simulink model "F1_Simulator"  (R2026a)
settings: Solver=VariableStepAuto  StopTime=260  MaxStep=0.01
values from neighbouring files (symbols this model uses):
  C = [C; C(1,:)]    [f1_corner_map.m]    (also in f1_lateral_tire_table.m = 1.3; f1_sector_map.m = C([true; hypot(diff(C(:,1)), diff(C(:,2))) > 1e-6], :); f1_sensitivity_sweep.m = {; f1_telemetry.m = C([true; hypot(diff(C(:,1)), diff(C(:,2))) > 1e-6], :))
  m = sU >= d0 & sU <= d1    [f1_corner_map.m]    (also in f1_sector_map.m = dC >= edM(k) & dC <= edM(k+1); f1_speed_profile.m = veh.m)
  normalX = -tangentY    [f1_finish_line_params.m]
  normalY = tangentX    [f1_finish_line_params.m]
  s = cumtrapz(tg, v)    [f1_internal_states.m]    (also in f1_track_animation.m = [0; cumsum(hypot(diff(x), diff(y)))]; f1_track_curvature.m = s_all(keepIdx))
  startX = track(1,1)    [f1_finish_line_params.m]
  startY = track(1,2)    [f1_finish_line_params.m]
  tangentX = dirVec(1)    [f1_finish_line_params.m]
  tangentY = dirVec(2)    [f1_finish_line_params.m]
  trackPsi = psi(idx)    [f1_load_raceline.m]    (also in f1_track_curvature.m = atan2(gradient(trackY), gradient(trackX)))
  trackVref = min(trackVref, vf)    [f1_speed_profile.m]
  trackX = x0    [f1_load_raceline.m]    (also in f1_track_curvature.m = x; silverstone_curvature.mat = [-563.032417564 -561.782952087 -560.539483404 -559.300900612)
  trackY = y0    [f1_load_raceline.m]    (also in f1_track_curvature.m = y; silverstone_curvature.mat = [-515.713759288 -514.151171661 -512.584488731 -511.014091481)
undefined symbols (not defined in the file or in its folder): fp_brk_bore, fp_brk_front, fp_brk_maxT, fp_brk_mu_k, fp_brk_pads, fp_brk_Rm, fp_CdA_corner, fp_CdA_straight, fp_eta_tr, fp_gears, fp_h_cg, fp_mu_brake, fp_mu_pk, fp_mu_trac, fp_N_diff, fp_rho, fp_rpm_dn, fp_rpm_lim_end, fp_rpm_lim_ini, fp_rpm_up, fp_track, pwr, veh
libraries: vehdynlibtire x4, autolibsharedcoupling x3, simulink x1, vehdynlibdriver x1, autolibsharedtransfixedgear x1, autolibshareddiff x1, autolibsharedmappedengines x1, autolibshared x1
(part 5 of 5)

== matlab function F1_Simulator/Vehicle Dynamics/Subsystem1/MATLAB Function3 ==
  data: TrqCmd_req input; TrqCmd output; EngSpd input; FzFL input; FzFR input; FzRL input; FzRR input; Re input; Gear input; fp_N_diff parameter; fp_eta_tr parameter; fp_gears parameter; fp_h_cg parameter; fp_mu_pk parameter; fp_mu_trac parameter; fp_rpm_lim_end parameter; fp_rpm_lim_ini parameter; fp_track parameter
function TrqCmd = f1_engine_cmd(TrqCmd_req, EngSpd, FzFL, FzFR, FzRL, FzRR, Re, Gear, fp_N_diff, fp_eta_tr, fp_gears, fp_h_cg, fp_mu_pk, fp_mu_trac, fp_rpm_lim_end, fp_rpm_lim_ini, fp_track)
% f1_engine_cmd  Engine torque command with (a) a grip limit and (b) a rev
% limiter. No states or loops: it cannot oscillate.
%
% (a) With an OPEN DIFFERENTIAL both wheels get the SAME torque, so the axle
%     can only push what the WEAKEST wheel holds:
%         T_axle <= 2*mu*min(FzRL, FzRR)*Re
%     (the inner wheel unloads in a corner, spins alone and the engine runs
%     into the rev limit). It is converted to ENGINE torque by dividing by the
%     total engine->axle ratio:
%       N_total = N_gear * N_diff * efficiency
%     The cut is made at the source (engine), not at the wheels, because
%     clipping the torque between two Torsional Compliance blocks leaves the
%     spring twisting without limit.
% (b) Above rpm_ini the torque ramps linearly down to 0 at rpm_fin. Without
%     it the engine map (held constant past 16000 rpm) would keep delivering
%     maximum torque at absurd speeds.
%
% Inputs
%   TrqCmd_req : torque requested from the engine [N*m] (the map reaches ~682)
%   EngSpd     : engine speed [rad/s]  (EngSpd output of the transmission)
%   FzFL..FzRR : vertical load of each wheel [N]. The rear ones limit the
%                torque; all 4 estimate how much grip the corner already uses
%                (friction circle)
%   Re         : effective wheel radius [m]
%   Gear       : engaged gear (2..8), from f1_shift_logic
% Output
%   TrqCmd     : command to the Mapped SI Engine [N*m]
%
% FRICTION CIRCLE: the grip available to push is what the tire has left after
% the lateral grip the corner already uses:
%     mu_x = min(mu, sqrt(mu_pk^2 - mu_y^2))
% with mu_y = Fy/sum(Fz) = |sum(Fz right) - sum(Fz left)| * track / (2*h_cg*sum(Fz))
% (the lateral load transfer measures the lateral force the car is making).
% With useFC = false the plain limit is recovered (mu_x = mu). No states or
% loops. If the torque oscillated, filter mu_y with a Transfer Fcn
% 1/(0.05 s + 1) in Simulink before it enters here.
%
% 7-SPEED GEARBOX (gears 2..8): ratio of the engaged gear = N vector of the
% transmission (at Re = 0.3515 m, from real telemetry).
%
% All shared values come from f1_vehicle_params.m through Parameter data
% (fp_*): change them there, not here.

Gvec     = [2 3 4 5 6 7 8];
Nvec     = fp_gears;
N_marcha = interp1(Gvec, Nvec, min(max(Gear, 2), 8), 'nearest');
N_diff   = fp_N_diff;          % final drive of the Active Differential
eta      = fp_eta_tr;          % transmission efficiency
mu       = fp_mu_trac;         % grip used by the limiter (real peak ~1.7)
rpm_ini  = fp_rpm_lim_ini;     % starts cutting
rpm_fin  = fp_rpm_lim_end;     % full cut
useFC    = true;               % friction circle (false = plain limit)
mu_pk    = fp_mu_pk;           % tire peak (Cy tables: 1.7 front / 1.8 rear)
mu_min   = 0.3;                % floor of mu_x: the push never goes fully to zero
track    = fp_track;           % [m] track (veh.track_f/r)
h_cg     = fp_h_cg;            % [m] = veh.cg_height (same h as the Vehicle Body load transfer)

% grip available to push (friction circle)
if useFC
    FzT  = max(FzFL + FzFR + FzRL + FzRR, 1);
    mu_y = min(abs((FzFR + FzRR) - (FzFL + FzRL)) * track / (2 * h_cg * FzT), mu_pk);
    mu_x = min(mu, max(sqrt(mu_pk^2 - mu_y^2), mu_min));
else
    mu_x = mu;
end

% (a) grip limit, as engine torque
Fz_w     = max(min(FzRL, FzRR), 0);   % weakest wheel (open differential)
Tmax_eje = 2 * mu_x * Fz_w * Re;
T_grip   = Tmax_eje / (N_marcha * N_diff * eta);

% (b) rev limiter
rpm = EngSpd * 30 / pi;
f   = min(1, max(0, (rpm_fin - rpm) / (rpm_fin - rpm_ini)));

TrqCmd = max(0, min(TrqCmd_req, T_grip)) * f;
end

== matlab function F1_Simulator/Pilot/MATLAB Function2 ==
  data: AccelCmd input; TrqCmd_req output; DecelCmd input; FzFL input; FzFR input; FzRL input; FzRR input; Re input; PrsFL output; PrsFR output; PrsRL output; PrsRR output; fp_brk_Rm parameter; fp_brk_bore parameter; fp_brk_front parameter; fp_brk_maxT parameter; fp_brk_mu_k parameter; fp_brk_pads parameter; fp_h_cg parameter; fp_mu_brake parameter; fp_mu_pk parameter; fp_track parameter
function [TrqCmd_req, PrsFL, PrsFR, PrsRL, PrsRR] = f1_pedals_to_cmd(AccelCmd, DecelCmd, FzFL, FzFR, FzRL, FzRR, Re, fp_brk_Rm, fp_brk_bore, fp_brk_front, fp_brk_maxT, fp_brk_mu_k, fp_brk_pads, fp_h_cg, fp_mu_brake, fp_mu_pk, fp_track)
% f1_pedals_to_cmd  Converts AccelCmd and DecelCmd from the Predictive Driver
% (0 to 1) into:
%   - TrqCmd_req : torque requested from the engine (goes to f1_engine_cmd,
%                  which applies the grip limit and the rev limit)
%   - PrsXX      : brake pressure of each wheel [Pa] (BrkPrs input of each
%                  Combined Slip Wheel with Brake type = Disc)
%
% The brake output is PRESSURE, not torque, because the BrkPrs port of the
% tire asks for it.
%
% Disc brake torque of the block (MathWorks documentation):
%     T = mu_kinetic * P * (pi*disk_abore^2/4) * Rm * num_pads
% so   P = T / Kdisc   with   Kdisc = mu_kinetic*pi*disk_abore^2/4*Rm*num_pads
% IMPORTANT: the disc parameters (brk.* in f1_vehicle_params.m) must be EQUAL
% to those of the Disc brake of the 4 tires.
%
% The brake is grip-limited in open loop (no feedback, cannot oscillate):
%     T_wheel <= mu_b * Fz_wheel * Re
%
% Inputs
%   AccelCmd, DecelCmd : normalized outputs of the Predictive Driver
%   FzFL..FzRR         : vertical load of each wheel [N]
%   Re                 : effective radius [m]
%
% FRICTION CIRCLE: when braking in a corner the tire is already spending
% lateral grip, so the brake limit drops:
%     mu_x = min(mu_b, sqrt(mu_pk^2 - mu_y^2)),   mu_y = Fy/sum(Fz)
% (mu_y is estimated from the lateral load transfer). With useFC = false the
% plain limit is recovered (mu_x = mu_b). No states.
%
% Shared values come from f1_vehicle_params.m through Parameter data (fp_*).

% --- powertrain and brake parameters ---
maxThrottleTrq = 682;            % N*m, maximum engine torque (end of the map)
maxBrakeTrq    = fp_brk_maxT;    % N*m, TOTAL brake torque on the 4 wheels
frontBias      = fp_brk_front;   % fraction of the braking on the front axle
mu_b           = fp_mu_brake;    % grip used by the brake limiter
useFC          = true;           % friction circle (false = plain limit)
mu_pk          = fp_mu_pk;       % tire peak
mu_min         = 0.3;            % floor of mu_x
track          = fp_track;       % [m] track
h_cg           = fp_h_cg;        % [m] = veh.cg_height (same h as the Vehicle Body load transfer)

% --- disc parameters (equal to those of each wheel block) ---
mu_k       = fp_brk_mu_k;        % mu_kinetic
disk_abore = fp_brk_bore;        % m
Rm         = fp_brk_Rm;          % m
num_pads   = fp_brk_pads;
Kdisc = mu_k * pi * disk_abore^2 / 4 * Rm * num_pads;   % N*m per Pa

acc = min(1, max(0, AccelCmd));
dec = min(1, max(0, DecelCmd));

% Throttle: fades out continuously when braking (no hard switch, to avoid
% zero crossings)
TrqCmd_req = maxThrottleTrq * acc * max(0, 1 - 5*dec);

% Brake: torque demand per wheel according to the split
demF = dec * maxBrakeTrq * frontBias / 2;          % each front wheel
demR = dec * maxBrakeTrq * (1 - frontBias) / 2;    % each rear wheel

% Grip available for braking (friction circle)
if useFC
    FzT  = max(FzFL + FzFR + FzRL + FzRR, 1);
    mu_y = min(abs((FzFR + FzRR) - (FzFL + FzRL)) * track / (2 * h_cg * FzT), mu_pk);
    mu_x = min(mu_b, max(sqrt(mu_pk^2 - mu_y^2), mu_min));
else
    mu_x = mu_b;
end

% Grip limit per wheel (as torque)
TFL = min(demF, mu_x * max(FzFL, 0) * Re);
TFR = min(demF, mu_x * max(FzFR, 0) * Re);
TRL = min(demR, mu_x * max(FzRL, 0) * Re);
TRR = min(demR, mu_x * max(FzRR, 0) * Re);

% Torque to pressure [Pa]
PrsFL = TFL / Kdisc;
PrsFR = TFR / Kdisc;
PrsRL = TRL / Kdisc;
PrsRR = TRR / Kdisc;

end

== matlab function F1_Simulator/Vehicle Dynamics/Subsystem1/MATLAB Function4 ==
  settings: updateMethod=DISCRETE
  data: vx input; Gear output; Re input; fp_N_diff parameter; fp_gears parameter; fp_rpm_dn parameter; fp_rpm_up parameter
function Gear = f1_shift_logic(vx, Re, fp_N_diff, fp_gears, fp_rpm_dn, fp_rpm_up)
% f1_shift_logic  Gear to engage according to the car speed (7-speed box, gears 2 to 8).
%
% Gear ratios (see f1_engine_cmd) taken from the real Silverstone telemetry:
% rpm / speed of each gear = median of the stable samples of that gear.
% 1st gear is not used (it is only for pulling away; the lap is a flying one).
%
% Shift rule (with hysteresis, taken from the telemetry: upshifts at ~10 900 rpm,
% median; 90 % between 10 300 and 11 400):
%   shift up   if rpm exceeds rpm_up
%   shift down if rpm falls below rpm_dn
% rpm_dn = 8500: after a downshift the rpm rise ~15-20 % (< 10 000), far from rpm_up.
%
% Inputs:  vx [m/s] longitudinal speed; Re [m] effective wheel radius.
% Output:  Gear (gear number, 2..8) -> Gear port of the transmission
%          and Gear input of f1_engine_cmd.
%
% It keeps one state (persistent) for the hysteresis. If the model uses a
% variable-step solver and repeated shifts show up, switch to a Memory block
% (feed Gear back).
%
% Shared values come from f1_vehicle_params.m through Parameter data (fp_*).

N_diff = fp_N_diff;
Nbox = fp_gears;           % gears 2..8 (at Re = 0.3515 m)
rpm_up = fp_rpm_up;
rpm_dn = fp_rpm_dn;

persistent g
if isempty(g)
    % initial gear: the lowest one with rpm <= rpm_up
    g = 7;
    for i = 1:7
        if max(vx, 0) / Re * Nbox(i) * N_diff * 30 / pi <= rpm_up
            g = i;
            break
        end
    end
end

rpm = max(vx, 0) / Re * Nbox(g) * N_diff * 30 / pi;
if rpm > rpm_up && g < 7
    g = g + 1;
elseif rpm < rpm_dn && g > 1
    g = g - 1;
end
Gear = g + 1;     % index 1..7 -> gear 2..8
end

== matlab function F1_Simulator/Pilot/MATLAB Function5 ==
  settings: updateMethod=DISCRETE
  data: carX input; RefPose output; carY input; carPsi input; trackX input; trackY input; trackPsi input; trackVref input; VelRef output
function [RefPose, VelRef] = f1_ref_pose(carX, carY, carPsi, trackX, trackY, trackPsi, trackVref)
% f1_ref_pose  Gives the Predictive Driver (Stanley) the point of the reference
% line closest to the car's CG, as a pose [Xref; Yref; Psiref].
%
% Why it exists: with "Vector input for poses" the block does NOT receive the
% whole track; it receives ONE reference pose per step, and the documentation
% says it must be "the point of the path closest to the CG". This function
% computes it.
%
% Design details:
%  1) The search runs in a window around the last index (as in
%     f1_locate_on_track): Silverstone passes close to itself (Wellington /
%     Village-The Loop) and a global search could latch onto another part of
%     the lap.
%  2) The car is projected onto the nearest segment (the vertex is not used):
%     the track has a point every 2 m, and the lateral error that Stanley sees
%     must not have "steps" of up to 1 m.
%  3) Psiref is delivered continuous with respect to the car's psi:
%         Psiref = carPsi + wrap(psiTrack - carPsi)
%     This way the heading error is always in (-pi, pi] and does not jump by
%     2*pi when crossing +-pi or when the lap closes.
%
% Inputs
%   carX, carY, carPsi : pose of the CG (CurrPose) [m, m, rad]
%   trackX, trackY     : reference line (silverstone_curvature.mat)
%   trackPsi           : track heading [rad] = atan2(gradient(trackY), gradient(trackX))
%   trackVref          : speed profile [m/s] (f1_speed_profile.m)
% Outputs
%   RefPose : [Xref, Yref, Psiref]  (1x3, row)
%   VelRef  : reference speed [m/s] at the closest point of the track

persistent lastIdx
N = numel(trackX);
if isempty(lastIdx)
    lastIdx = 1;          % the car starts at the finish line (first point)
end

window = 50;              % +-50 points = +-100 m at 2 m/point
idx = mod((lastIdx-1-window):(lastIdx-1+window), N) + 1;
dx = trackX(idx) - carX;
dy = trackY(idx) - carY;
[~, k] = min(dx.^2 + dy.^2);
i0 = idx(k);
lastIdx = i0;

iN = mod(i0, N) + 1;      % next vertex (circular)
iP = mod(i0 - 2, N) + 1;  % previous vertex (circular)

% Projection onto the two segments that touch the closest vertex
[tA, xA, yA, dA] = projSeg(carX, carY, trackX(i0), trackY(i0), trackX(iN), trackY(iN));
[tB, xB, yB, dB] = projSeg(carX, carY, trackX(iP), trackY(iP), trackX(i0), trackY(i0));

if dA <= dB
    Xref = xA;  Yref = yA;
    psiTrack = trackPsi(i0) + tA * wrapPi(trackPsi(iN) - trackPsi(i0));
else
    Xref = xB;  Yref = yB;
    psiTrack = trackPsi(iP) + tB * wrapPi(trackPsi(i0) - trackPsi(iP));
end

Psiref = carPsi + wrapPi(psiTrack - carPsi);

RefPose = [Xref, Yref, Psiref];   % ROW 1x3: this is what "Pose Routing" of the Predictive Driver requires
VelRef  = trackVref(i0);          % speed profile at the closest point
end

function [t, px, py, d2] = projSeg(cx, cy, ax, ay, bx, by)
% Projects (cx,cy) onto the segment A-B; t in [0,1]
abx = bx - ax;  aby = by - ay;
L2  = abx*abx + aby*aby;
if L2 < 1e-9
    t = 0;
else
    t = ((cx - ax)*abx + (cy - ay)*aby) / L2;
    t = min(1, max(0, t));
end
px = ax + t*abx;
py = ay + t*aby;
d2 = (cx - px)^2 + (cy - py)^2;
end

function a = wrapPi(a)
a = mod(a + pi, 2*pi) - pi;
end

== matlab function F1_Simulator/Vehicle Dynamics/Subsystem1/MATLAB Function6 ==
  settings: updateMethod=DISCRETE
  data: vx input; FExt output; r input; fp_CdA_corner parameter; fp_CdA_straight parameter; fp_rho parameter
function FExt = f1_aero_active(vx, r, fp_CdA_corner, fp_CdA_straight, fp_rho)
%F1_AERO_ACTIVE  Straight mode of the active aerodynamics (step 1: drag only).
%
%   Inputs:  vx = longitudinal speed [m/s]   (xdot output of the Vehicle Body)
%            r  = yaw rate [rad/s]           (r output of the Vehicle Body)
%   Output:  FExt = [Fx Fy Fz] [N] -> FExt port of the Vehicle Body
%
%   The Vehicle Body already computes the drag of the corner mode (Cd 0.73,
%   Af 1.5). In straight mode the real drag is lower, so the DIFFERENCE is
%   injected here as a forward force:
%       dFx = 0.5*rho*vx^2*(CdA_corner - CdA_straight)
%
%   CdA_straight is a CALIBRATION value (no published 2026 data).
%   Shared values come from f1_vehicle_params.m through Parameter data (fp_*).

CdA_curva = fp_CdA_corner;     % m^2, the Vehicle Body one (aero.Cd_corner * aero.Af)
CdA_recta = fp_CdA_straight;   % m^2, to calibrate with f1_measure_accel
rho       = fp_rho;            % kg/m^3 (288.15 K, 101325 Pa)

% Hysteresis to avoid switching constantly: decided with the approximate
% lateral acceleration ay = r*vx
ay_in  = 3;                 % m/s^2: below this it enters straight mode
ay_out = 6;                 % m/s^2: above this it goes back to corner mode
vx_min = 40;                % m/s: not active at low speed

persistent recta
if isempty(recta), recta = false; end

ay = abs(r * vx);
if recta
    if ay > ay_out || vx < vx_min, recta = false; end
else
    if ay < ay_in && vx > vx_min,  recta = true;  end
end

if recta
    dFx = 0.5 * rho * vx^2 * (CdA_curva - CdA_recta);
else
    dFx = 0;
end

FExt = [dFx 0 0];
end

== matlab function F1_Simulator/Vehicle Dynamics/Subsystem1/MATLAB Function1 ==
  data: FxFL input; FwF output; FxFR input
function FwF = fcn(FxFL, FxFR)
FwF = [FxFL, FxFR];
end

== matlab function F1_Simulator/Vehicle Dynamics/Subsystem1/MATLAB Function ==
  data: Vx input; VxFL output; Vy input; r input; track_f input; track_r input; a input; b input; VxFR output; VxRL output; VxRR output; VyFL output; VyFR output; VyRL output; VyRR output
function [VxFL,VxFR,VxRL,VxRR,VyFL,VyFR,VyRL,VyRR] = fcn(Vx,Vy,r,track_f,track_r,a,b)
VxFL = Vx - r*track_f/2;
VxFR = Vx + r*track_f/2;
VxRL = Vx - r*track_r/2;
VxRR = Vx + r*track_r/2;
VyFL = Vy + r*a;
VyFR = Vy + r*a;
VyRL = Vy - r*b;
VyRR = Vy - r*b;
end

== matlab function F1_Simulator/Vehicle Dynamics/Subsystem1/MATLAB Function2 ==
  data: FxRL input; FwR output; FxRR input
function FwR = fcn(FxRL, FxRR)
FwR = [FxRL, FxRR];
end

== matlab function F1_Simulator/LapTimer/MATLAB Function ==
  settings: updateMethod=DISCRETE
  data: carX input; lapCount output; carY input; simTime input; startX input; startY input; tangentX input; tangentY input; normalX input; normalY input; currentLapTime output; lastLapTime output
function [lapCount, currentLapTime, lastLapTime] = f1_lap_timer(carX, carY, simTime, ...
    startX, startY, tangentX, tangentY, normalX, normalY)
% f1_lap_timer  Detects crossings of the finish line and keeps the lap record.
%
% Inputs (all scalars):
%   carX, carY          - current car position
%   simTime             - current simulation time
%   startX, startY      - finish line point (from f1_finish_line_params.m)
%   tangentX, tangentY  - direction of travel at the finish line (unit vector)
%   normalX, normalY    - perpendicular to the direction of travel
%
% Outputs:
%   lapCount       - number of completed laps
%   currentLapTime - time elapsed since the last crossing (lap in progress,
%                    useful for a live display)
%   lastLapTime    - time of the last completed lap (it stays fixed until the
%                    next crossing - the lap time table is built from this
%                    after the simulation)

persistent lapCountP lastCrossTimeP lastTangSignP lastLapTimeP isFirstCall
if isempty(lapCountP)
    lapCountP = 0;
    lastCrossTimeP = 0;
    lastLapTimeP = 0;
    lastTangSignP = 0;
    isFirstCall = true;
end

% Local coordinates relative to the finish line: how far the car has advanced
% (tangential) and how far it is displaced sideways (normal)
dx = carX - startX;
dy = carY - startY;
tangDist = dx*tangentX + dy*tangentY;
perpDist = dx*normalX + dy*normalY;
currentTangSign = sign(tangDist);

tol = 30;        % [m] lateral tolerance width; avoids confusing the line with
% another distant point of the circuit that, by geometry,
% lies near the same extended imaginary line
gracePeriod = 2; % [s] no crossing counts before this time has passed since the
% last crossing (or since the start). Without it, a car that
% starts exactly at tangDist = 0 triggers a false "crossing"
% on the first step, because sign(0) = 0 is treated as
% "before the finish line".

if isFirstCall
    % On the first call only the initial sign is stored - the car starts right
    % at the finish line, and that must not count as a lap
    lastTangSignP = currentTangSign;
    isFirstCall = false;
else
    timeSinceLastCross = simTime - lastCrossTimeP;
    crossed = (lastTangSignP <= 0) && (currentTangSign > 0) && ...
        (abs(perpDist) < tol) && (timeSinceLastCross > gracePeriod);
    if crossed
        lastLapTimeP = simTime - lastCrossTimeP;
        lastCrossTimeP = simTime;
        lapCountP = lapCountP + 1;
    end
    lastTangSignP = currentTangSign;
end

lapCount = lapCountP;
currentLapTime = simTime - lastCrossTimeP;
lastLapTime = lastLapTimeP;
end
